simulink model "cartpole_sim_OL"  (R2026a)
settings: Solver=ode45  MaxStep=1e-1  RelTol=1e-12  AbsTol=1e-12
settings Model: Creator=santi  LastModifiedBy=elkin

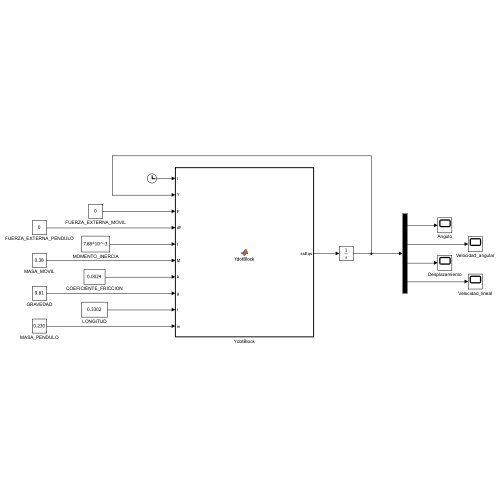
[thumbnail: Simulink's stored preview of the top-level diagram]
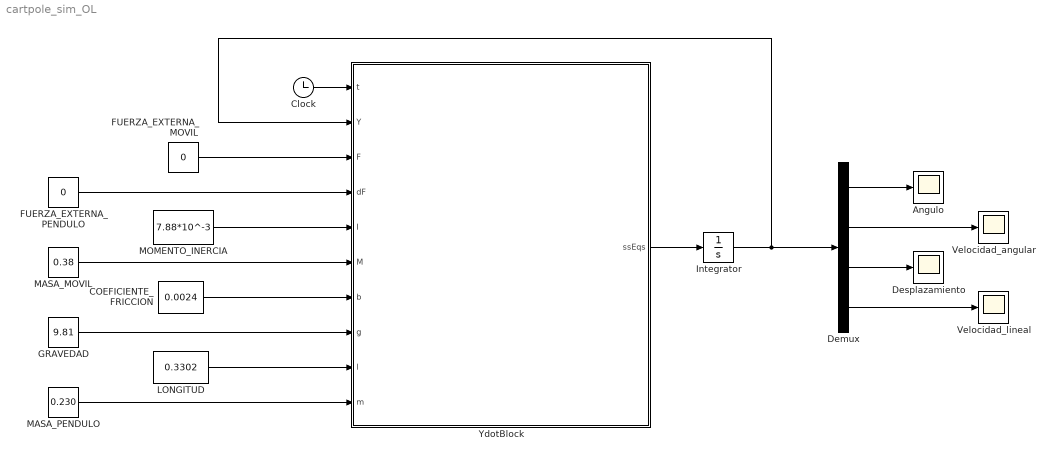
== system cartpole_sim_OL ==
  Angulo : Scope
      settings: ActiveDisplayYMinimum=-1  ActiveDisplayYMaximum=1
  COEFICIENTE_FRICCION : Constant  Value=0.0024
  Clock : Clock
  Demux : Demux
  Desplazamiento : Scope
      settings: ActiveDisplayYMinimum=-1  ActiveDisplayYMaximum=1  DataLoggingVariableName=ScopeData2
  FUERZA_EXTERNA_MOVIL : Constant  Value=0
  FUERZA_EXTERNA_PENDULO : Constant  Value=0
  GRAVEDAD : Constant  Value=9.81
  Integrator : Integrator
  LONGITUD : Constant  Value=0.3302
  MASA_MOVIL : Constant  Value=0.38
  MASA_PENDULO : Constant  Value=0.230
  MOMENTO_INERCIA : Constant  Value=7.88*10^-3
  Velocidad_angular : Scope
      settings: ActiveDisplayYMinimum=-1  ActiveDisplayYMaximum=1
  Velocidad_lineal : Scope
      settings: ActiveDisplayYMinimum=-1  ActiveDisplayYMaximum=1  DataLoggingVariableName=ScopeData3
  YdotBlock : MATLAB Function  TreatAsAtomicUnit=on
  wires:
  FUERZA_EXTERNA_MOVIL/1 -> YdotBlock/3(F)
  FUERZA_EXTERNA_PENDULO/1 -> YdotBlock/4(dF)
  MOMENTO_INERCIA/1 -> YdotBlock/5(I)
  MASA_MOVIL/1 -> YdotBlock/6(M)
  COEFICIENTE_FRICCION/1 -> YdotBlock/7(b)
  GRAVEDAD/1 -> YdotBlock/8(g)
  LONGITUD/1 -> YdotBlock/9(l)
  MASA_PENDULO/1 -> YdotBlock/10(m)
  YdotBlock/1(ssEqs) -> Integrator/1
  Integrator/1 -> Demux/1, YdotBlock/2(Y)
  Clock/1 -> YdotBlock/1(t)
  Demux/1 -> Angulo/1
  Demux/2 -> Velocidad_angular/1
  Demux/3 -> Desplazamiento/1
  Demux/4 -> Velocidad_lineal/1

== matlab function cartpole_sim_OL/YdotBlock ==
  data: t input; ssEqs output; Y input size=[4 1]; F input; dF input; I input; M input; b input; g input; l input; m input
function ssEqs = YdotBlock(t,Y,F,dF,I,M,b,g,l,m)
%#codegen

%    This function was generated by the Symbolic Math Toolbox version 25.1.
%    01-Nov-2026 18:24:22

% t = complex(t);  % if required to enforce complex operations
% Y = complex(Y);  % if required to enforce complex operations
% F = complex(F);  % if required to enforce complex operations
% dF = complex(dF);  % if required to enforce complex operations
% I = complex(I);  % if required to enforce complex operations
% M = complex(M);  % if required to enforce complex operations
% b = complex(b);  % if required to enforce complex operations
% g = complex(g);  % if required to enforce complex operations
% l = complex(l);  % if required to enforce complex operations
% m = complex(m);  % if required to enforce complex operations
t2 = I.*m;
t3 = Y(1);
t4 = Y(2);
t5 = Y(4);
t6 = l.^2;
t7 = m.^2;
t8 = I.*M;
t9 = cos(t3);
t10 = sin(t3);
t11 = t4.^2;
t13 = M.*m.*t6;
t14 = t6.*t7;
t12 = t9.^2;
t15 = t12.*t14;
t16 = -t15;
t17 = t2+t8+t13+t14+t16;
t18 = 1.0./t17;
ssEqs = [t4;l.*t18.*(M.*dF.*t9+F.*m.*t9+g.*t7.*t10-b.*m.*t5.*t9+M.*g.*m.*t10-l.*t7.*t9.*t10.*t11);t5;-t18.*(I.*dF-F.*I+I.*b.*t5-F.*m.*t6+dF.*m.*t6+b.*m.*t5.*t6-dF.*m.*t6.*t12-g.*t9.*t10.*t14+l.*t2.*t10.*t11+l.^3.*t7.*t10.*t11)];
end
